simulink model "Pay_load"  (R2025a)
settings: Solver=ode4  StartTime=0.0  StopTime=1  FixedStep=0.001  RelTol=1e-3
values from neighbouring files (symbols this model uses):
  angle1_init = [0;0;0.3]    [param.m]
  angle2_init = [0;0;0.3]    [param.m]
  angle3_init = [0;0;0.3]    [param.m]
  angle4_init = [0;0;0.3]    [param.m]
  joint_matrix = [r1; r2; r3; r4]    [param.m]
  m1 = 1    [param.m]
  m2 = 1    [param.m]
  m3 = 1    [param.m]
  m4 = 1    [param.m]
  mL = 2    [param.m]
  P = block.DialogPrm(1).Data    [Load_dynamic.m]    (also in param.m = struct())
  p1_init = pL_init + RL_init*r1 - l1*e1    [param.m]
  p2_init = pL_init + RL_init*r2 - l2*e2    [param.m]
  p3_init = pL_init + RL_init*r3 - l3*e3    [param.m]
  p4_init = pL_init + RL_init*r4 - l4*e4    [param.m]
  r1 = [ 0.25; -0.20; -0.45]    [param.m]
  r2 = [-0.50; -0.40; -0.15]    [param.m]
  r3 = [-0.50;  0.40;  0.15]    [param.m]
  r4 = [ 0.50;  0.40;  0.00]    [param.m]
  xL_init = [pL_init; vL_init; angle_L_init; omega_L_init]    [param.m]
(part 3 of 3)

== matlab function Pay_load/UAV4 Controller/Subsystem1/Position Controller/MATLAB Function1 ==
  data: dei input; eta_ei input; d_eta_d_dei input; ei input; eij input; d_ij input; Ei output; eta_eij input; d_eta_d_eij input
function Ei = fcn(dei, eta_ei, d_eta_d_dei, ei, eij, d_ij, eta_eij, d_eta_d_eij)

    Ei = zeros(3,1);

    A = d_eta_d_dei * sqrt(d_eta_d_dei) * ei;
    
    B = zeros(3,1);
    for i = 1:3
        B = B + 2*eta_eij(i)*d_eta_d_eij(i)*eij(((i-1)*3+1):(i*3),1)/d_ij(i);
    end

    Ei = A + B;

end

== matlab function Pay_load/UAV4 Controller/Subsystem1/Subsystem/MATLAB Function ==
  data: pi input; vi input; ui output; alpha_pi input; alpha_pi_dot input; Ei input; cable_tension input; delta_i input; rho_mi input; xL input; z2i output; ubar_i output; delta_i_dot output; rho_mi_dot output; m parameter; ri parameter
function [ui, z2i, ubar_i, delta_i_dot, rho_mi_dot] = ...
    Velocity_Control_41_44(pi, vi, alpha_pi, alpha_pi_dot, Ei, ...
                          cable_tension, delta_i, rho_mi, xL, m, ri)
    %#codegen
    % Vector inputs: 3x1
    % mi, delta_i, rho_mi: scalar
    
    K2i       = 3.15;
    epsilon_i = 0.1;
    
    n_delta     = 0.15;
    sigma_delta = 0.05;
    
    n_rho_m     = 0.1;
    sigma_rho_m = 0.01;
    
    assert(m > 0);
    
    ez = [0; 0; 1];
    
    z2i = vi - alpha_pi;
    z2_sq = z2i.' * z2i;
    
    %% Equation (42)
    pL = xL(1:3,1); phi_L = xL(7,1); theta_L = xL(8,1); psi_L = xL(9,1);

    RL = [cos(theta_L)*cos(psi_L), sin(phi_L)*sin(theta_L)*cos(psi_L) - cos(phi_L)*sin(psi_L), cos(phi_L)*sin(theta_L)*cos(psi_L) + sin(phi_L)*sin(psi_L);
          cos(theta_L)*sin(psi_L), sin(phi_L)*sin(theta_L)*sin(psi_L) + cos(phi_L)*cos(psi_L), cos(phi_L)*sin(theta_L)*sin(psi_L) - sin(phi_L)*cos(psi_L);
          -sin(theta_L), sin(phi_L)*cos(theta_L), cos(phi_L)*cos(theta_L)];

    qi = RL.'*(pL + RL*ri - pi)/norm(pL + RL*ri - pi);

    fCablePred_i = RL*qi*(cable_tension.'*qi);

    ubar_i = Ei - alpha_pi_dot ...
             + 9.81 * ez ...
             + K2i * z2i ...
             + delta_i * z2i / sqrt(z2_sq + epsilon_i^2) ...
             + fCablePred_i / m;
    
    %% Equation (41)
    ubar_sq = ubar_i.' * ubar_i;
    A = ubar_sq * rho_mi^2;
    
    ui = z2i * A / sqrt(z2_sq * A + epsilon_i^2);
    
    %% Equation (43)
    delta_i_dot = n_delta * z2_sq ...
                  / sqrt(z2_sq + epsilon_i^2) ...
                  - sigma_delta * delta_i;
    
    %% Equation (44)
    rho_mi_dot = n_rho_m * (z2i.' * ubar_i) ...
                - sigma_rho_m * rho_mi;

end

== matlab function Pay_load/UAV4 Controller/Subsystem1/Subsystem/MATLAB Function1 ==
  data: ui input; Fi output; psi_di input; angle_di_prev input; angle_di output size=[3,1]; valid output
function [Fi, angle_di, valid] = ...
    Desired_Attitude_85_87(ui, psi_di, angle_di_prev)
%#codegen
% ui, angle_di_prev: 3x1
% psi_di, Fi: scalar
% valid: boolean

Fmin = 1e-8;

Fi = norm(ui);
angle_di = angle_di_prev;
valid = false;

% Khi ui gan 0, huong luc khong xac dinh.
% Giu goc dat truoc do, khong chia cho Fi.
if Fi <= Fmin
    return;
end

% Mien Euler bay thang dang su dung:
% |phi_di| < pi/2, |theta_di| < pi/2.
% assert(ui(3) > 0);

sphi = (ui(1)*sin(psi_di) ...
        - ui(2)*cos(psi_di)) / Fi;

% Chi chan sai so lam tron cua asin.
sphi = min(1.0, max(-1.0, sphi));

phi_di = asin(sphi);

theta_di = atan2( ...
    ui(1)*cos(psi_di) + ui(2)*sin(psi_di), ui(3));

angle_di = [phi_di; theta_di; psi_di];
valid = true;

end

== matlab function Pay_load/Subsystem3/UAV4/MATLAB Function1 ==
  data: tau input; omega_dot output; omega input; Iv parameter
function omega_dot = fcn(tau, omega, Iv)

    omega_dot = zeros(3,1);

    omega_dot = Iv \ (tau - cross(omega, Iv*omega));

end

== matlab function Pay_load/MATLAB Function ==
  data: u input; angle_L_dot output; angle_L input
function angle_L_dot = fcn(u, angle_L)

    angle_L_dot = zeros(3,1);

    phi_L = angle_L(1); theta_L = angle_L(2); psi_L = angle_L(3);

    Gamma_L = [1, sin(phi_L)*tan(theta_L), cos(phi_L)*tan(theta_L);
                0, cos(phi_L), -sin(phi_L);
                0, sin(phi_L)/cos(theta_L), cos(phi_L)/cos(theta_L)];

    angle_L_dot = Gamma_L*u;

end

== matlab function Pay_load/MATLAB Function1 ==
  data: t input; pdL output
function pdL = fcn(t)

    pdL = zeros(3,1);

    xdL = 0.2*t - 0.35;
    ydL = 3.5*sin(0.15*t);
    zdL = -0.2*t + 0.01*sin(25*t) - 1.5;

    pdL = [xdL; ydL; zdL];

end

== matlab function Pay_load/MATLAB Function2 ==
  data: t input; pd1 output; pd2 output; pd3 output; pd4 output
function [pd1, pd2, pd3, pd4] = Generate_pdi(t)
%#codegen
% Vi tri dat cua 4 UAV theo quy dao trong bai bao.
% Quy uoc: truc z huong xuong.

%% Tham so
li = 2.5;       % Chieu dai day [m]
varphi = 0.35;
lookahead = 2;  % Thoi gian nhin truoc [s]

% Diem gan day trong he toa do tai
r1 = [ 0.25; -0.20; -0.45];
r2 = [-0.50; -0.40; -0.15];
r3 = [-0.50;  0.40;  0.15];
r4 = [ 0.50;  0.40;  0.00];

%% Vi tri tai dat tai thoi diem t
pdL = [0.2*t - 0.35;
       3.5*sin(0.15*t);
       -0.2*t + 0.01*sin(25*t) - 1.5];

%% Vi tri tai dat tai thoi diem t + 2
tf = t + lookahead;

pdL_future = [0.2*tf - 0.35;
              3.5*sin(0.15*tf);
              -0.2*tf + 0.01*sin(25*tf) - 1.5];

%% Huong day dat: tu UAV den diem gan day tren tai
Delta = pdL - pdL_future;
D = norm(Delta);

assert(D > 1e-8, 'Khong xac dinh duoc huong day dat.');

edi = [varphi*Delta(1)/D;
       varphi*Delta(2)/D;
       sqrt(1 - varphi^2 + varphi^2*(Delta(3)/D)^2)];

%% Vi tri dat UAV
% angle_dL = [0;0;0] => R_dL = eye(3)
% pdi = pdL + R_dL*ri - li*edi

pd1 = pdL + r1 - li*edi;
pd2 = pdL + r2 - li*edi;
pd3 = pdL + r3 - li*edi;
pd4 = pdL + r4 - li*edi;

end

== matlab function Pay_load/Subsystem/UAV1/MATLAB Function3 ==
  data: thrust input; a_free output; angular input
function a_free = UAV_FreeAcceleration(thrust, angular)

    m = 1;

    phi   = angular(1);
    theta = angular(2);
    psi   = angular(3);
    
    % Cot thu ba cua ma tran quay R: R*[0;0;1]
    b3 = [cos(psi)*sin(theta)*cos(phi) + sin(psi)*sin(phi);
          sin(psi)*sin(theta)*cos(phi) - cos(psi)*sin(phi);
          cos(theta)*cos(phi)];
    
    assert(m > 0);
    
    a_free = [0;0;9.81] - (thrust/m)*b3;
end

== matlab function Pay_load/Subsystem1/UAV2/MATLAB Function3 ==
  data: thrust input; a_free output; angular input
function a_free = UAV_FreeAcceleration(thrust, angular)

    m = 1;

    phi   = angular(1);
    theta = angular(2);
    psi   = angular(3);
    
    % Cot thu ba cua ma tran quay R: R*[0;0;1]
    b3 = [cos(psi)*sin(theta)*cos(phi) + sin(psi)*sin(phi);
          sin(psi)*sin(theta)*cos(phi) - cos(psi)*sin(phi);
          cos(theta)*cos(phi)];
    
    assert(m > 0);
    
    a_free = [0;0;9.81] - (thrust/m)*b3;
end

== matlab function Pay_load/Subsystem2/UAV3/MATLAB Function3 ==
  data: thrust input; a_free output; angular input
function a_free = UAV_FreeAcceleration(thrust, angular)

    m = 1;

    phi   = angular(1);
    theta = angular(2);
    psi   = angular(3);
    
    % Cot thu ba cua ma tran quay R: R*[0;0;1]
    b3 = [cos(psi)*sin(theta)*cos(phi) + sin(psi)*sin(phi);
          sin(psi)*sin(theta)*cos(phi) - cos(psi)*sin(phi);
          cos(theta)*cos(phi)];
    
    assert(m > 0);
    
    a_free = [0;0;9.81] - (thrust/m)*b3;
end

== matlab function Pay_load/Subsystem3/UAV4/MATLAB Function3 ==
  data: thrust input; a_free output; angular input
function a_free = UAV_FreeAcceleration(thrust, angular)

    m = 1;

    phi   = angular(1);
    theta = angular(2);
    psi   = angular(3);
    
    % Cot thu ba cua ma tran quay R: R*[0;0;1]
    b3 = [cos(psi)*sin(theta)*cos(phi) + sin(psi)*sin(phi);
          sin(psi)*sin(theta)*cos(phi) - cos(psi)*sin(phi);
          cos(theta)*cos(phi)];
    
    assert(m > 0);
    
    a_free = [0;0;9.81] - (thrust/m)*b3;
end

== matlab function Pay_load/MATLAB Function3 ==
  data: xL input; dxL output size=[12,1]; pD12 input size=[12,1]; vD12 input size=[12,1]; aFree12 input size=[12,1]; fD12 output; P parameter
function [dxL, fD12] = Load_Cable_Dynamics( ...
    xL, pD12, vD12, aFree12, P)
%#codegen
% Khai bao P la Parameter trong MATLAB Function.
%
% xL      : 12x1 [pL; vL; EulerL; omegaL_body]
% pD12    : 12x1 [p1; p2; p3; p4]
% vD12    : 12x1 [v1; v2; v3; v4]
% aFree12 : 12x1 gia toc UAV chua co luc day
%
% dxL     : 12x1 dao ham trang thai tai
% fD12    : 12x1 luc day tac dung len 4 UAV, he the gioi

pD = reshape(pD12,    3,4);
vD = reshape(vD12,    3,4);
a0 = reshape(aFree12, 3,4);

pL    = xL(1:3);
vL    = xL(4:6);
angle = xL(7:9);
omega = xL(10:12);

R = rotationZYX(angle);

B    = zeros(4,6);
D    = zeros(4,4);
rhs  = zeros(4,1);
sAll = zeros(3,4);

for i = 1:4
    ri = P.r(:,i);

    % Vector tu UAV den diem treo tren tai, he the gioi
    s = pL + R*ri - pD(:,i);
    s2 = s.'*s;

    assert(s2 > 1e-12);

    % Van toc tuong doi hai dau day
    sd = vL + R*cross(omega,ri) - vD(:,i);

    % Sai lech rang buoc chieu dai day
    c    = 0.5*(s2 - P.ell(i)^2);
    cdot = s.'*sd;

    b = sd.'*sd ...
        + s.'*R*cross(omega,cross(omega,ri));

    correction = 2*P.zeta*P.wn*cdot + P.wn^2*c;

    B(i,:) = [s.', -s.'*R*skew3(ri)];
    D(i,i) = s2/P.mD(i);

    rhs(i) = s.'*a0(:,i) - b - correction;
    sAll(:,i) = s;
end

% He phuong trinh dong luc hoc va rang buoc 4 day
ML = blkdiag(P.mL*eye(3), P.JL);

QL = [P.mL*[0;0;P.g];
      -cross(omega,P.JL*omega)];

K = [ML, B.';
     B, -D];

solution = K \ [QL; rhs];

aL       = solution(1:3);
omegaDot = solution(4:6);
lambda   = solution(7:10);

% Luc day THUC tac dung len UAV, he the gioi
fD = zeros(3,4);
for i = 1:4
    fD(:,i) = sAll(:,i)*lambda(i);
end
fD12 = reshape(fD,12,1);

% Bien doi van toc goc than -> dao ham goc Euler
phi   = angle(1);
theta = angle(2);

assert(abs(cos(theta)) > 1e-6);

Gamma = [1, sin(phi)*tan(theta), cos(phi)*tan(theta);
         0, cos(phi),           -sin(phi);
         0, sin(phi)/cos(theta), cos(phi)/cos(theta)];

dxL = [vL;
       aL;
       Gamma*omega;
       omegaDot];
end

function R = rotationZYX(angle)
phi   = angle(1);
theta = angle(2);
psi   = angle(3);

cp = cos(phi);   sp = sin(phi);
ct = cos(theta); st = sin(theta);
cy = cos(psi);   sy = sin(psi);

R = [cy*ct, cy*st*sp-sy*cp, cy*st*cp+sy*sp;
     sy*ct, sy*st*sp+cy*cp, sy*st*cp-cy*sp;
     -st,   ct*sp,          ct*cp];
end

function S = skew3(v)
S = [0,    -v(3),  v(2);
     v(3),  0,   -v(1);
    -v(2),  v(1),  0];
end

== matlab function Pay_load/PayLoad Controller/Equation (18) ==
  data: eta_eL output; deri output; EL output; pL input; alpha_pL output; pdL input; pdL_dot input; t input
function [eta_eL, deri, EL, alpha_pL] = fcn(pL, pdL, pdL_dot, t)

    K1L = 3.55;

    deL = norm(pL - pdL);
    EL = 1/deL*(pL - pdL);

    Omega_dHL = (7.8 - 0.2)*exp(-0.4*t) + 0.2;
    Omega_dHL_dot = -0.4*7.6*exp(-0.4*t);

    deri = Omega_dHL^2/(Omega_dHL - deL)^2;
    
    eta_eL = (Omega_dHL * deL)/(Omega_dHL - deL);

    alpha_pL = (EL*(Omega_dHL - deL)^2/Omega_dHL^2)*((-deL^2/(Omega_dHL - deL)^2)*Omega_dHL_dot - K1L*eta_eL) + pdL_dot;
end
